simulink subsystem "Slosh_Axis"  (R2026a)
settings: Solver=VariableStepAuto
settings Model: Creator=asing  LastModifiedBy=asing

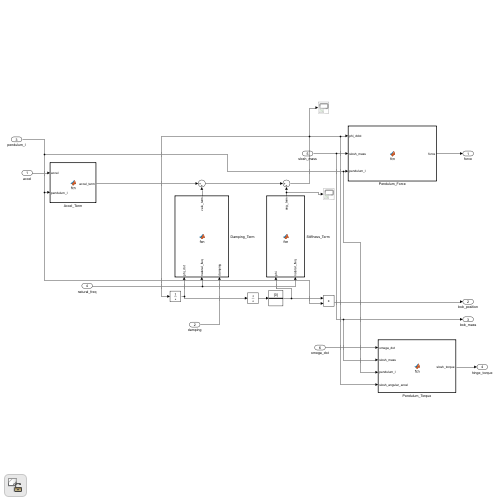
[thumbnail: Simulink's stored preview of the top-level diagram]
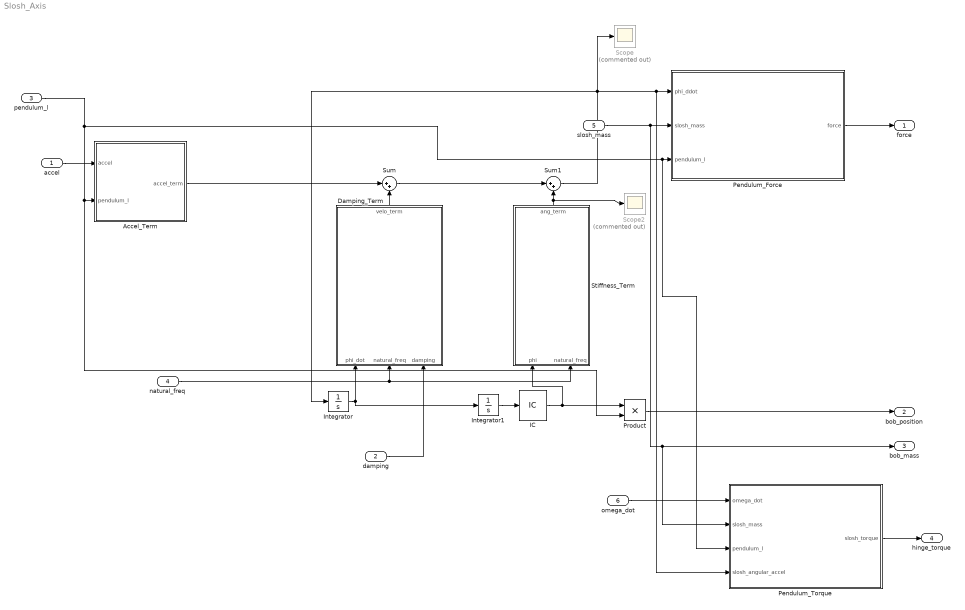
== system Slosh_Axis ==
  accel : Inport
  damping : Inport  Port=2
  pendulum_l : Inport  Port=3
  natural_freq : Inport  Port=4
  slosh_mass : Inport  Port=5
  omega_dot : Inport  Port=6
  Accel_Term : MATLAB Function  TreatAsAtomicUnit=on
  Damping_Term : MATLAB Function  TreatAsAtomicUnit=on
  IC : InitialCondition  Value=0
  Integrator : Integrator
  Integrator1 : Integrator
  Pendulum_Force : MATLAB Function  TreatAsAtomicUnit=on
  Pendulum_Torque : MATLAB Function  TreatAsAtomicUnit=on
  Product : Product
  Scope : Scope  Commented=on
      settings: ActiveDisplayYMinimum=-22308.19804574037  ActiveDisplayYMaximum=11892.944291168513  DataLoggingVariableName=ScopeData28
  Scope2 : Scope  Commented=on
      settings: ActiveDisplayYMinimum=-120826.17462841458  ActiveDisplayYMaximum=34452.37997376953  DataLoggingVariableName=ScopeData46
  Stiffness_Term : MATLAB Function  TreatAsAtomicUnit=on
  Sum : Sum  Inputs=|++
  Sum1 : Sum  Inputs=|++
  force : Outport
  bob_position : Outport  Port=2
  bob_mass : Outport  Port=3
  hinge_torque : Outport  Port=4
  wires:
  accel/1 -> Accel_Term/1(accel)
  pendulum_l/1 -> Pendulum_Force/3(pendulum_l), Pendulum_Torque/3(pendulum_l), Product/2, Accel_Term/2(pendulum_l)
  Integrator/1 -> Integrator1/1, Damping_Term/1(phi_dot)
  Damping_Term/1(velo_term) -> Sum/2
  natural_freq/1 -> Stiffness_Term/2(natural_freq), Damping_Term/2(natural_freq)
  damping/1 -> Damping_Term/3(damping)
  Sum/1 -> Sum1/1
  Stiffness_Term/1(ang_term) -> Sum1/2, Scope2/1
  Accel_Term/1(accel_term) -> Sum/1
  Sum1/1 -> Scope/1, Pendulum_Force/1(phi_ddot), Pendulum_Torque/4(slosh_angular_accel), Integrator/1
  slosh_mass/1 -> Pendulum_Torque/2(slosh_mass), bob_mass/1, Pendulum_Force/2(slosh_mass)
  Pendulum_Force/1(force) -> force/1
  IC/1 -> Stiffness_Term/1(phi), Product/1
  Integrator1/1 -> IC/1
  Product/1 -> bob_position/1
  omega_dot/1 -> Pendulum_Torque/1(omega_dot)
  Pendulum_Torque/1(slosh_torque) -> hinge_torque/1

== matlab function Slosh_Axis/Accel_Term ==
  data: accel input; accel_term output; pendulum_l input
function accel_term = fcn(accel, pendulum_l)

accel_term = -accel / pendulum_l;

end

== matlab function Slosh_Axis/Stiffness_Term ==
  data: phi input; ang_term output; natural_freq input
function ang_term = fcn(phi, natural_freq)

ang_term = -natural_freq^2 * phi;

end

== matlab function Slosh_Axis/Damping_Term ==
  data: phi_dot input; velo_term output; natural_freq input; damping input
function velo_term = fcn(phi_dot, natural_freq,damping)

velo_term = -2 * damping * natural_freq * phi_dot;
end

== matlab function Slosh_Axis/Pendulum_Force ==
  data: phi_ddot input; force output; slosh_mass input; pendulum_l input
function force = fcn(phi_ddot, slosh_mass, pendulum_l)
% Force of the pendulum on the tank, beyond the rigid propellant already in
% the vehicle mass: -m1 * y_ddot, y = l*phi the body-frame bob displacement
% (phi_ddot = -a/l - w^2 phi - 2 zeta w phi_dot). Sign was +m1*y_ddot,
% which added m1 to the lateral inertia instead of removing it.
force = -slosh_mass * pendulum_l * phi_ddot;
end

== matlab function Slosh_Axis/Pendulum_Torque ==
  data: omega_dot input; slosh_torque output; slosh_mass input; pendulum_l input; slosh_angular_accel input
function slosh_torque = fcn(omega_dot, slosh_mass, pendulum_l, slosh_angular_accel)
% Per-pendulum torque removed. A pendulum analog (SP-106, Dodge 2000,
% SLOSH-ML) is a point mass on a frictionless hinge: it has no rotational
% inertia of its own and transmits no moment through the hinge. The old
% -m*l^2*(omega_dot - phi_ddot) term added a fictitious inertia m*l^2 and a
% hinge moment. The liquid rigid-body inertia (the analog's I0) is carried
% by the CG/MOI tables. Inputs kept for the
% subsystem interface.
slosh_torque = 0 * omega_dot;
end
